simulink model "EV_Truck_Model"  (R2022b)
settings: Solver=FixedStepAuto  StartTime=0  StopTime=26553  FixedStep=0.1  RelTol=1e-3
model workspace (MAT data in the model file):
  ADAS_MaxAccel = 2
  ADAS_MaxDecel = 2.5
  Adas_on_off = 0
  Batt_cap_ah : Simulink.Parameter (value not decoded)
  Batt_rist_r0 : Simulink.Parameter (value not decoded)
  Batt_soc_s0 : Simulink.Parameter (value not decoded)
  Batt_volt_v0 : Simulink.Parameter (value not decoded)
  Motor_eff_100 : Simulink.Parameter (value not decoded)
  Motor_eff_190 : Simulink.Parameter (value not decoded)
  Motor_eff_95 : Simulink.Parameter (value not decoded)
  Motor_rpm_100 : Simulink.Parameter (value not decoded)
  Motor_rpm_190 : Simulink.Parameter (value not decoded)
  Motor_rpm_95 : Simulink.Parameter (value not decoded)
  Motor_torque_pos_100 : Simulink.Parameter (value not decoded)
  Motor_torque_pos_190 : Simulink.Parameter (value not decoded)
  Motor_torque_pos_95 : Simulink.Parameter (value not decoded)
  Motor_trq_190 : Simulink.Parameter (value not decoded)
  Motor_trq_95 : Simulink.Parameter (value not decoded)
  Sim_step = 0.1
  Test_DriveCycle = 0
  Trans_ratio = 6.142
  Veh_cog_fx = 1.69543
  Veh_cog_h = 0.605887
  Veh_cog_rx = 2.11956
  Veh_diff = 6.7
  Veh_whl_crr = 0.01
  Veh_whl_k = 180000
  Veh_whl_radius = 0.35
symbols that are objects in the model workspace (value not decoded): Motor_eff_100, Motor_eff_190, Motor_eff_95, Motor_rpm_100, Motor_rpm_190, Motor_rpm_95, Motor_torque_pos_100, Motor_torque_pos_190, Motor_torque_pos_95, Motor_trq_190, Motor_trq_95
undefined symbols (not defined in the file): Batt_soc_init, canChannel, Elec_aux_sw, Elec_rgn_sw, Power_option, speed, time, Veh_mass
libraries: batteryecm_lib x170, simulink x14, canmsglib x9, canlib x7, autolibshared x5, nesl_utility x4, fl_lib x3, drivingvehiclecontroller x3, hdlsllib x3, sim3dlib x1, sim3dautolib x1, vrlib x1
(part 2 of 11)

== system EV_Truck_Model/Accumulator System ==
  note: Voltage-Capacity Relationship
      | 100% 3.65V
      | 99% 3.4V
      | 98% 3.32V
      | 97% 3.3V
      | Linear
      | 50% 3.2V
      | 20% 3.1V
      | 15% 3.0V
      | 10% 2.8V
      | 5% 2.5V
      | 0% 2.0V
      | Singel Cell Internal Resistance: 3mOhm
      | Parallel Cell Internal Resistance: 0.5mOhm
      | http://hf-gotion.com/products/case5/7.html
  Current : Inport
  2-D Lookup Table : Lookup_n-D  Commented=on  BreakpointsForDimension1=[1:3]  BreakpointsForDimension2=[1:3]  InternalRulePriority=Speed  RndMeth=Simplest
      settings: InputPortMap=u0,u1
  Battery (Table-Based) : batteryecm_lib/Battery (Table-Based)  Tag={'toolbox/physmod/battery/shared_library/m/batteryecm_lib_parts';'Battery__Table_Based_/A123/ALM12V7.xml'}  Commented=through  SOC_vec=[0 0.01 0.02 0.03 0.04 0.05 0.06 0.07 0.08 0.09 0.1 0.11 0.12 0.13 0.14 0.15 0.16 0.17 0.18 0.19 0.2 0.21 0.22 0.23 0.24 0.25 0.26 0.27 0.28 0.29 0.3 0.31 0.32 0.33 0.34 0.35 0.36 0.37 0.38 0.39 0.4 0.41 0.42 0.43 0.44 0.45 0.46 0.47 0.48 0.49 0.5 0.51 0.52 0.53 0.54 0.55 0.56 0.57 0.58 0.59 0.6 0.61 0.62 0.63 0.64 0.65 0.66 0.67 0.68 0.69 0.7 0.71 0.72 0.73 0.74 0.75 0.76 0.77 0.78 0.79 0.8 0.81 0.82 0.83 0.84 0.85 0.86 0.87 0.88 0.89 0.9 0.91 0.92 0.93 0.94 0.95 0.96 0.97 0.98 0.99 1]  T_dependence=simscape.enum.tablebattery.temperature_dependence.yes  prm_dir=simscape.enum.tablebattery.prm_dir.noCurrentDirectionality  T_vec=[0 25 45] degC  V0_mat=[8.05812 7.90952 10.84524;8.40413 8.34439 12.167;8.75015 8.77925 12.48061;9.09617 9.21411 12.63926;9.44219 9.64898 12.66062;9.7882 10.08384 12.66196;10.13422 10.74357 12.71107;10.48024 11.30381 12.78816;10.82626 11.63268 12.79883;11.17301 11.93821 12.78814;11.4915 12.15298 12.76631;11.73964 12.3273 12.75774;11.93281 12.43261 12.76614;12.03376 12.50816 12.77788;12.15804 12.57594 12.79587;12.26092 12.61755 12.81552;12.35763 12.64457 12.83633;12.46264 12.68224 12.84719;12.54135 12.71382 12.85759;12.61973 12.74201 12.87378;12.68064 12.76384 12.89165;12.7273 12.7798 12.90334;12.75019 12.8011 12.91442;12.7795 12.81807 12.92545;12.79476 12.83474 12.93649;12.80199 12.84972 12.94845;12.79988 12.86401 12.96057;12.8064 12.87896 12.97362;12.81314 12.89327 12.9873;12.81905 12.90705 13.00097;12.8231 12.92025 13.01743;12.83144 12.93293 13.03449;12.84056 12.94496 13.05153;12.84748 12.95422 13.06837;12.8514 12.96347 13.08315;12.85351 12.97316 13.09593;12.86138 12.98357 13.10749;12.87252 12.99397 13.11297;12.87348 13.00292 13.1193;12.87448 13.00978 13.12225;12.88062 13.01665 13.12493;12.88615 13.02351 13.1275;12.89358 13.02933 13.12903;12.90102 13.03559 13.13047;12.90646 13.04185 13.1317;12.91023 13.04811 13.13261;12.91373 13.05484 13.1336;12.91916 13.06156 13.13482;12.92679 13.06811 13.13582;12.93442 13.07393 13.13682;12.93761 13.07931 13.13785;12.93879 13.08459 13.14019;12.94047 13.08888 13.1426;12.94372 13.09316 13.14505;12.94697 13.09745 13.14506;12.95275 13.10191 13.14506;12.95871 13.10663 13.14507;12.96447 13.11149 13.14537;12.97023 13.11625 13.14712;12.97671 13.12077 13.14887;12.98396 13.1253 13.15078;12.9912 13.12947 13.15349;12.99846 13.13339 13.15917;13.00592 13.13718 13.16486;13.0098 13.142 13.17126;13.01315 13.14683 13.1789;13.01642 13.15338 13.18676;13.0194 13.1606 13.19727;13.0225 13.16782 13.20775;13.03012 13.17504 13.21901;13.03927 13.18103 13.23221;13.04842 13.18612 13.24601;13.05758 13.19115 13.25559;13.06673 13.19583 13.26268;13.07323 13.20057 13.26837;13.07926 13.20546 13.27148;13.08529 13.21036 13.27459;13.09132 13.21551 13.27817;13.10058 13.22106 13.28185;13.11119 13.22814 13.28528;13.12181 13.23521 13.28448;13.13279 13.24229 13.2834;13.14332 13.24921 13.28542;13.14826 13.25386 13.28855;13.15276 13.25892 13.29055;13.15658 13.26397 13.29097;13.15965 13.26903 13.29534;13.1637 13.27459 13.29849;13.16904 13.2803 13.29921;13.17556 13.28425 13.29987;13.18215 13.2873 13.30304;13.18702 13.29077 13.30748;13.18906 13.29423 13.31134;13.19472 13.29701 13.31689;13.20216 13.30359 13.32162;13.20682 13.31175 13.33363;13.21832 13.31809 13.34341;13.22486 13.34117 13.3682;13.25687 13.37591 13.4231;13.3584 13.50696 13.59952;13.73658 14.69171 14.24081] V  V0_vec=[7.90952 8.34439 8.77925 9.21411 9.64898 10.08384 10.74357 11.30381 11.63268 11.93821 12.15298 12.3273 12.43261 12.50816 12.57594 12.61755 12.64457 12.68224 12.71382 12.74201 12.76384 12.7798 12.8011 12.81807 12.83474 12.84972 12.86401 12.87896 12.89327 12.90705 12.92025 12.93293 12.94496 12.95422 12.96347 12.97316 12.98357 12.99397 13.00292 13.00978 13.01665 13.02351 13.02933 13.03559 13.04185 13.04811 13.05484 13.06156 13.06811 13.07393 13.07931 13.08459 13.08888 13.09316 13.09745 13.10191 13.10663 13.11149 13.11625 13.12077 13.1253 13.12947 13.13339 13.13718 13.142 13.14683 13.15338 13.1606 13.16782 13.17504 13.18103 13.18612 13.19115 13.19583 13.20057 13.20546 13.21036 13.21551 13.22106 13.22814 13.23521 13.24229 13.24921 13.25386 13.25892 13.26397 13.26903 13.27459 13.2803 13.28425 13.2873 13.29077 13.29423 13.29701 13.30359 13.31175 13.31809 13.34117 13.37591 13.50696 14.69171] V  V_range=[9 Inf] V  R0_mat=[0.24852 0.16316 0.37407;0.27167 0.15014 0.44119;0.29483 0.13711 0.39874;0.31798 0.12409 0.33945;0.34114 0.11107 0.253;0.36429 0.09804 0.17297;0.38744 0.09898 0.137;0.4106 0.09406 0.11837;0.43375 0.07751 0.0969;0.45706 0.07197 0.08022;0.47423 0.06587 0.06407;0.47611 0.06364 0.05484;0.46604 0.05937 0.05112;0.43592 0.0557 0.04879;0.41518 0.05497 0.04766;0.39502 0.05305 0.04722;0.3785 0.05058 0.04739;0.36725 0.05063 0.04645;0.34844 0.05036 0.04531;0.33707 0.04999 0.0448;0.32097 0.04932 0.045;0.30505 0.04837 0.04454;0.28497 0.04827 0.04408;0.2684 0.04798 0.04361;0.25118 0.04766 0.04314;0.23446 0.04729 0.04289;0.21678 0.04694 0.04266;0.20301 0.0471 0.04269;0.19098 0.04724 0.0429;0.1805 0.04736 0.0431;0.17153 0.04745 0.04377;0.16488 0.04751 0.04456;0.15901 0.04755 0.04534;0.15295 0.04741 0.04605;0.14764 0.04727 0.04643;0.1423 0.04726 0.04659;0.13996 0.04731 0.04663;0.13837 0.04736 0.04628;0.13485 0.04731 0.0463;0.13134 0.04714 0.04596;0.12898 0.04697 0.04558;0.1265 0.0468 0.04516;0.12564 0.04664 0.04461;0.12479 0.04662 0.04405;0.1235 0.04659 0.04344;0.12161 0.04657 0.04278;0.11961 0.04658 0.04214;0.11837 0.04659 0.04165;0.11809 0.04657 0.04112;0.11781 0.04651 0.0406;0.11651 0.04644 0.0401;0.11476 0.04636 0.03973;0.11322 0.04622 0.03938;0.11237 0.04607 0.03905;0.11152 0.04593 0.03846;0.11122 0.04582 0.03787;0.11069 0.04573 0.03729;0.11008 0.04565 0.03668;0.10947 0.04556 0.03617;0.10916 0.04546 0.03567;0.10918 0.04535 0.03524;0.10919 0.04524 0.03503;0.10922 0.04511 0.03515;0.10933 0.04499 0.03527;0.10866 0.04502 0.03552;0.10787 0.04505 0.03591;0.10706 0.04519 0.03633;0.10611 0.04538 0.03685;0.10519 0.04556 0.03735;0.10529 0.04574 0.03794;0.10605 0.04585 0.03887;0.10682 0.04586 0.04006;0.10758 0.04586 0.0408;0.10835 0.04585 0.04126;0.10839 0.04585 0.04147;0.10829 0.04585 0.04134;0.10819 0.04586 0.0412;0.10809 0.0459 0.04113;0.10886 0.046 0.04108;0.10997 0.04618 0.041;0.11107 0.04637 0.04018;0.11233 0.04655 0.03922;0.11356 0.04673 0.03886;0.11359 0.04676 0.03865;0.11341 0.04683 0.03842;0.11294 0.04689 0.03823;0.11231 0.04695 0.03846;0.1122 0.04704 0.03796;0.11241 0.04714 0.03717;0.11291 0.04696 0.03641;0.11346 0.0466 0.03639;0.11363 0.04626 0.0365;0.11258 0.04592 0.0362;0.11218 0.04538 0.0359;0.11216 0.04507 0.03525;0.11038 0.04454 0.03533;0.11007 0.04279 0.03431;0.1059 0.04194 0.03432;0.09933 0.03873 0.03411;0.09302 0.03651 0.038;0.07895 0.07068 0.04545] Ohm  R0_vec=[0.16316 0.15014 0.13711 0.12409 0.11107 0.09804 0.09898 0.09406 0.07751 0.07197 0.06587 0.06364 0.05937 0.0557 0.05497 0.05305 0.05058 0.05063 0.05036 0.04999 0.04932 0.04837 0.04827 0.04798 0.04766 0.04729 0.04694 0.0471 0.04724 0.04736 0.04745 0.04751 0.04755 0.04741 0.04727 0.04726 0.04731 0.04736 0.04731 0.04714 0.04697 0.0468 0.04664 0.04662 0.04659 0.04657 0.04658 0.04659 0.04657 0.04651 0.04644 0.04636 0.04622 0.04607 0.04593 0.04582 0.04573 0.04565 0.04556 0.04546 0.04535 0.04524 0.04511 0.04499 0.04502 0.04505 0.04519 0.04538 0.04556 0.04574 0.04585 0.04586 0.04586 0.04585 0.04585 0.04585 0.04586 0.0459 0.046 0.04618 0.04637 0.04655 0.04673 0.04676 0.04683 0.04689 0.04695 0.04704 0.04714 0.04696 0.0466 0.04626 0.04592 0.04538 0.04507 0.04454 0.04279 0.04194 0.03873 0.03651 0.07068] Ohm  R0_dis_mat=[.0117, .0085, .009; .011, .0085, .009; .0114, .0087, .0092; .0107, .0082, .0088; .0107, .0083, .0091; .0113, .0085, .0089; .0116, .0085, .0089] % Parameter not set Ohm  R0_dis_vec=[.0085, .0085, .0087, .0082, .0083, .0085, .0085] % Parameter not set Ohm  R0_ch_mat=[.0117, .0085, .009; .011, .0085, .009; .0114, .0087, .0092; .0107, .0082, .0088; .0107, .0083, .0091; .0113, .0085, .0089; .0116, .0085, .0089] % Parameter not set Ohm  R0_ch_vec=[.0085, .0085, .0087, .0082, .0083, .0085, .0085] % Parameter not set Ohm  AH=4.911 hr*A  prm_leak=simscape.enum.tablebattery.prm_leak.disabled  Rleak_vec=[8000, 7000, 6000] % Parameter not set Ohm  Rleak=7e3 % Parameter not set Ohm  extrapolation_option=simscape.enum.extrapolation.nearest  SOC_port=simscape.enum.tablebattery.enable.no  prm_dyn=simscape.enum.tablebattery.prm_dyn.off  R1_mat=[.0109, .0029, .0013; .0069, .0024, .0012; .0047, .0026, .0013; .0034, .0016, .001; .0033, .0023, .0014; .0033, .0018, .0011; .0028, .0017, .0011] % Parameter not set Ohm  R1_vec=[.0029, .0024, .0026, .0016, .0023, .0018, .0017] % Parameter not set Ohm  tau1_mat=[20, 36, 39; 31, 45, 39; 109, 105, 61; 36, 29, 26; 59, 77, 67; 40, 33, 29; 25, 39, 33] % Parameter not set s  tau1_vec=[36, 45, 105, 29, 77, 33, 39] % Parameter not set s  R2_mat=[.0109, .0029, .0013; .0069, .0024, .0012; .0047, .0026, .0013; .0034, .0016, .001; .0033, .0023, .0014; .0033, .0018, .0011; .0028, .0017, .0011] % Parameter not set Ohm  R2_vec=[.0029, .0024, .0026, .0016, .0023, .0018, .0017] % Parameter not set Ohm  tau2_mat=[20, 36, 39; 31, 45, 39; 109, 105, 61; 36, 29, 26; 59, 77, 67; 40, 33, 29; 25, 39, 33] % Parameter not set s  tau2_vec=[36, 45, 105, 29, 77, 33, 39] % Parameter not set s  R3_mat=[.0109, .0029, .0013; .0069, .0024, .0012; .0047, .0026, .0013; .0034, .0016, .001; .0033, .0023, .0014; .0033, .0018, .0011; .0028, .0017, .0011] % Parameter not set Ohm  R3_vec=[.0029, .0024, .0026, .0016, .0023, .0018, .0017] % Parameter not set Ohm  tau3_mat=[20, 36, 39; 31, 45, 39; 109, 105, 61; 36, 29, 26; 59, 77, 67; 40, 33, 29; 25, 39, 33] % Parameter not set s  tau3_vec=[36, 45, 105, 29, 77, 33, 39] % Parameter not set s  R4_mat=[.0109, .0029, .0013; .0069, .0024, .0012; .0047, .0026, .0013; .0034, .0016, .001; .0033, .0023, .0014; .0033, .0018, .0011; .0028, .0017, .0011] % Parameter not set Ohm  R4_vec=[.0029, .0024, .0026, .0016, .0023, .0018, .0017] % Parameter not set Ohm  tau4_mat=[20, 36, 39; 31, 45, 39; 109, 105, 61; 36, 29, 26; 59, 77, 67; 40, 33, 29; 25, 39, 33] % Parameter not set s  tau4_vec=[36, 45, 105, 29, 77, 33, 39] % Parameter not set s  R5_mat=[.0109, .0029, .0013; .0069, .0024, .0012; .0047, .0026, .0013; .0034, .0016, .001; .0033, .0023, .0014; .0033, .0018, .0011; .0028, .0017, .0011] % Parameter not set Ohm  R5_vec=[.0029, .0024, .0026, .0016, .0023, .0018, .0017] % Parameter not set Ohm  tau5_mat=[20, 36, 39; 31, 45, 39; 109, 105, 61; 36, 29, 26; 59, 77, 67; 40, 33, 29; 25, 39, 33] % Parameter not set s  tau5_vec=[36, 45, 105, 29, 77, 33, 39] % Parameter not set s  prm_fade=simscape.enum.tablebattery.prm_fade.tableN  N0=100 % Parameter not set  dV0=0 % Parameter not set  dR0=0 % Parameter not set  dAH=0 % Parameter not set  dRleak=0 % Parameter not set  dR1=0 % Parameter not set  dR2=0 % Parameter not set  dR3=0 % Parameter not set  dR4=0 % Parameter not set  dR5=0 % Parameter not set  N0vec=[1 76 151 226 301 376 451 526 601 676 751 826 901 976 1051 1126 1201 1276 1351 1426 1501 1576 1651 1726 1801 1876 1951 2026 2101 2176 2251 2326 2401 2476 2551 2626 2701 2776 2851 2926 3001 3076 3151 3226 3301 3376 3451 3526 3601 3676 3751 3826 3901 3976 4051 4126 4201 4276 4351 4426 4501 4576 4651 4726 4801 4876 4951 5026 5101 5176 5251 5326 5401 5476 5551 5626 5701 5776 5851 5926 6001 6076 6151 6226 6301 6376 6451 6526 6601 6676 6751 6826 6901 6976 7051 7126 7201 7276 7351]  Tfadevec=[298.15, 323.15] % Parameter not set K  dV0vec=[0 -2.2983 -4.5967 -6.895 -8.189 -8.4451 -8.8012 -9.0094 -9.1038 -9.1836 -9.2343 -9.282 -9.3297 -9.3564 -9.3673 -9.3782 -9.3891 -9.402 -9.4162 -9.4327 -9.4491 -9.4624 -9.4766 -9.4917 -9.4989 -9.5047 -9.5093 -9.5145 -9.5202 -9.5259 -9.531 -9.5361 -9.5412 -9.5463 -9.5514 -9.557 -9.5622 -9.5672 -9.5722 -9.5771 -9.5822 -9.5878 -9.5934 -9.599 -9.6046 -9.6114 -9.6185 -9.6256 -9.6327 -9.6397 -9.6463 -9.651 -9.6557 -9.6605 -9.6652 -9.67 -9.6747 -9.6803 -9.6857 -9.6908 -9.6959 -9.701 -9.7064 -9.7127 -9.7189 -9.7252 -9.7314 -9.738 -9.7446 -9.7511 -9.7577 -9.7643 -9.767 -9.7695 -9.772 -9.7748 -9.7798 -9.7848 -9.7896 -9.7948 -9.8002 -9.8056 -9.811 -9.8162 -9.8181 -9.8205 -9.8232 -9.8259 -9.8291 -9.836 -9.843 -9.8499 -9.8569 -9.8644 -9.872 -9.8797 -9.8867 -9.8926 -9.8986]  dR0vec=[0 0 0 0 0 0 0 0 0 0 0 0 0 0 0 0 0 0 0 0 0 0 0 0 0 0 0 0 0 0 0 0 0 0 0 0 0 0 0 0 0 0 0 0 0 0 0 0 0 0 0 0 0 0 0 0 0 0 0 0 0 0 0 0 0 0 0 0 0 0 0 0 0 0 0 0 0 0 0 0 0 0 0 0 0 0 0 0 0 0 0 0 0 0 0 0 0 0 0] % Parameter assumed  dAHvec=[0 -0.285 -0.57 -0.855 -1.14 -1.427 -1.826 -2.226 -2.625 -2.962 -3.266 -3.569 -3.873 -4.157 -4.409 -4.662 -4.914 -5.167 -5.421 -5.719 -6.017 -6.316 -6.632 -6.968 -7.304 -7.613 -7.858 -8.103 -8.349 -8.589 -8.804 -9.02 -9.236 -9.452 -9.668 -9.906 -10.145 -10.384 -10.623 -10.862 -11.083 -11.291 -11.499 -11.707 -11.914 -12.118 -12.3 -12.482 -12.664 -12.846 -13.015 -13.14 -13.265 -13.39 -13.515 -13.64 -13.766 -13.913 -14.061 -14.21 -14.358 -14.506 -14.664 -14.846 -15.027 -15.209 -15.391 -15.582 -15.772 -15.963 -16.154 -16.345 -16.424 -16.497 -16.569 -16.65 -16.796 -16.943 -17.09 -17.252 -17.423 -17.594 -17.765 -17.93 -17.987 -18.044 -18.1 -18.157 -18.226 -18.373 -18.52 -18.668 -18.815 -18.974 -19.134 -19.294 -19.438 -19.562 -19.686]  dRleakvec=[0, 0, 0] % Parameter not set  dR1vec=[0, 0, 0] % Parameter not set  dR2vec=[0, 0, 0] % Parameter not set  dR3vec=[0, 0, 0] % Parameter not set  dR4vec=[0, 0, 0] % Parameter not set  dR5vec=[0, 0, 0] % Parameter not set  dV0mat=[0, 0; 0, 0; 0, 0] % Parameter not set  dR0mat=[0, 0; 0, 0; 0, 0] % Parameter not set  dAHmat=[0, 0; 0, 0; 0, 0] % Parameter not set  dRleakmat=[0, 0; 0, 0; 0, 0] % Parameter not set  dR1mat=[0, 0; 0, 0; 0, 0] % Parameter not set  dR2mat=[0, 0; 0, 0; 0, 0] % Parameter not set  dR3mat=[0, 0; 0, 0; 0, 0] % Parameter not set  dR4mat=[0, 0; 0, 0; 0, 0] % Parameter not set  dR5mat=[0, 0; 0, 0; 0, 0] % Parameter not set  prm_age_modeling=simscape.enum.tablebattery.prm_age_modeling.equation  storage_dt_age_vec=[0] % Parameter not set d  storage_T_age_vec=[273] % Parameter not set K  prm_age_OCV=simscape.enum.tablebattery.prm_age_OCV.OCV  OCV_age=0.9 % Parameter not set  SOC_age=0.6 % Parameter not set  prm_age_resistance=simscape.enum.tablebattery.prm_age.disabled  OCV_scaling_age_resistance=2.2134e6 % Parameter not set  OCV_offset_age_resistance=1.632e6 % Parameter not set  temp_exp_age_resistance=0.515833569 % Parameter not set V  t_exp_age_resistance=0.75 % Parameter not set  T_age_vec_resistance=[273.15, 298.15, 323.15] % Parameter not set K  dt_age_vec_resistance=[90, 180, 270, 360] % Parameter not set d  dR0_age_vec=[0, 0, 0] % Parameter not set  t_meas_dR0_age=100 % Parameter not set d  dR0_age_mat=[0, 0, 0; 0, 0, 0; 0, 0, 0; 0, 0, 0] % Parameter not set  prm_age_capacity=simscape.enum.tablebattery.prm_age.disabled  OCV_scaling_age_capacity=1.5097e07 % Parameter not set  OCV_offset_age_capacity=8.3625e06 % Parameter not set  temp_exp_age_capacity=0.6011 % Parameter not set V  t_exp_age_capacity=0.75 % Parameter not set  T_age_vec_capacity=[273.15, 298.15, 323.15] % Parameter not set K  dt_age_vec_capacity=[90, 180, 270, 360] % Parameter not set d  dAH_age_vec=[0, 0, 0] % Parameter not set  t_meas_dAH_age=100 % Parameter not set d  dAH_age_mat=[0, 0, 0; 0, 0, 0; 0, 0, 0; 0, 0, 0] % Parameter not set  thermal_port=simscape.enum.thermaleffects.omit  temperature=298.15 % Parameter not set K  thermal_mass=756 % Parameter assumed J/K  i_specify=off  i_priority=None  i=0 A  i_nominal_specify=off  i_nominal_unit=A  i_nominal_value=1  v_specify=off  v_priority=None  v=0 V  v_nominal_specify=off  v_nominal_unit=V  v_nominal_value=1  stateOfCharge_specify=off  stateOfCharge_priority=High  stateOfCharge=1  stateOfCharge_nominal_specify=off  stateOfCharge_nominal_unit=1  stateOfCharge_nominal_value=1  num_cycles_specify=off  num_cycles_priority=High  num_cycles=0  num_cycles_nominal_specify=off  num_cycles_nominal_unit=1  num_cycles_nominal_value=1  cell_temperature_specify=off  cell_temperature_priority=High  cell_temperature=298.15 K  cell_temperature_nominal_specify=off  cell_temperature_nominal_unit=K  cell_temperature_nominal_value=1
      settings: AttributesFormatString=A123:ALM12V7  InternalSimscapePortConfiguration="{\"Bottom\":[],\"Left\":[{\"id\":\"p\",\"label\":\"+\",\"type\":\"foundation.electrical.electrical\"}],\"Right\":[{\"id\":\"n\",\"label\":\"-\",\"type\":\"foundation.electrical.electrical\"}],\"Top\":[]}"
  Battery Pack : Subsystem
  Battery1 : batteryecm_lib/Battery (Table-Based)  Commented=on  SOC_vec=Batt_soc_s0  T_dependence=simscape.enum.tablebattery.temperature_dependence.no  prm_dir=simscape.enum.tablebattery.prm_dir.noCurrentDirectionality  T_vec=[293] K  V0_mat=[2, 3, 3.2, 3.25, 3.25, 3.3, 3.3, 3.3, 3.35, 3.5] V  V0_vec=Batt_volt_v0 V  V_range=[0, inf] V  R0_mat=[15] mOhm  R0_vec=Batt_rist_r0 mOhm  R0_dis_mat=[.0117, .0085, .009; .011, .0085, .009; .0114, .0087, .0092; .0107, .0082, .0088; .0107, .0083, .0091; .0113, .0085, .0089; .0116, .0085, .0089] Ohm  R0_dis_vec=[.0085, .0085, .0087, .0082, .0083, .0085, .0085] Ohm  R0_ch_mat=[.0117, .0085, .009; .011, .0085, .009; .0114, .0087, .0092; .0107, .0082, .0088; .0107, .0083, .0091; .0113, .0085, .0089; .0116, .0085, .0089] Ohm  R0_ch_vec=[.0085, .0085, .0087, .0082, .0083, .0085, .0085] Ohm  AH=Batt_cap_ah A*hr  prm_leak=simscape.enum.tablebattery.prm_leak.disabled  Rleak_vec=[8000, 7000, 6000] Ohm  Rleak=7e3 Ohm  extrapolation_option=simscape.enum.extrapolation.nearest  SOC_port=simscape.enum.tablebattery.enable.no  prm_dyn=simscape.enum.tablebattery.prm_dyn.off  R1_mat=[.0109, .0029, .0013; .0069, .0024, .0012; .0047, .0026, .0013; .0034, .0016, .001; .0033, .0023, .0014; .0033, .0018, .0011; .0028, .0017, .0011] Ohm  R1_vec=[.0029, .0024, .0026, .0016, .0023, .0018, .0017] Ohm  tau1_mat=[20, 36, 39; 31, 45, 39; 109, 105, 61; 36, 29, 26; 59, 77, 67; 40, 33, 29; 25, 39, 33] s  tau1_vec=[36, 45, 105, 29, 77, 33, 39] s  R2_mat=[.0109, .0029, .0013; .0069, .0024, .0012; .0047, .0026, .0013; .0034, .0016, .001; .0033, .0023, .0014; .0033, .0018, .0011; .0028, .0017, .0011] Ohm  R2_vec=[.0029, .0024, .0026, .0016, .0023, .0018, .0017] Ohm  tau2_mat=[20, 36, 39; 31, 45, 39; 109, 105, 61; 36, 29, 26; 59, 77, 67; 40, 33, 29; 25, 39, 33] s  tau2_vec=[36, 45, 105, 29, 77, 33, 39] s  R3_mat=[.0109, .0029, .0013; .0069, .0024, .0012; .0047, .0026, .0013; .0034, .0016, .001; .0033, .0023, .0014; .0033, .0018, .0011; .0028, .0017, .0011] Ohm  R3_vec=[.0029, .0024, .0026, .0016, .0023, .0018, .0017] Ohm  tau3_mat=[20, 36, 39; 31, 45, 39; 109, 105, 61; 36, 29, 26; 59, 77, 67; 40, 33, 29; 25, 39, 33] s  tau3_vec=[36, 45, 105, 29, 77, 33, 39] s  R4_mat=[.0109, .0029, .0013; .0069, .0024, .0012; .0047, .0026, .0013; .0034, .0016, .001; .0033, .0023, .0014; .0033, .0018, .0011; .0028, .0017, .0011] Ohm  R4_vec=[.0029, .0024, .0026, .0016, .0023, .0018, .0017] Ohm  tau4_mat=[20, 36, 39; 31, 45, 39; 109, 105, 61; 36, 29, 26; 59, 77, 67; 40, 33, 29; 25, 39, 33] s  tau4_vec=[36, 45, 105, 29, 77, 33, 39] s  R5_mat=[.0109, .0029, .0013; .0069, .0024, .0012; .0047, .0026, .0013; .0034, .0016, .001; .0033, .0023, .0014; .0033, .0018, .0011; .0028, .0017, .0011] Ohm  R5_vec=[.0029, .0024, .0026, .0016, .0023, .0018, .0017] Ohm  tau5_mat=[20, 36, 39; 31, 45, 39; 109, 105, 61; 36, 29, 26; 59, 77, 67; 40, 33, 29; 25, 39, 33] s  tau5_vec=[36, 45, 105, 29, 77, 33, 39] s  prm_fade=simscape.enum.tablebattery.prm_fade.disabled  N0=100  dV0=0  dR0=0  dAH=0  dRleak=0  dR1=0  dR2=0  dR3=0  dR4=0  dR5=0  N0vec=[100, 200, 300]  Tfadevec=[298.15, 323.15] K  dV0vec=[0, 0, 0]  dR0vec=[0, 0, 0]  dAHvec=[0, 0, 0]  dRleakvec=[0, 0, 0]  dR1vec=[0, 0, 0]  dR2vec=[0, 0, 0]  dR3vec=[0, 0, 0]  dR4vec=[0, 0, 0]  dR5vec=[0, 0, 0]  dV0mat=[0, 0; 0, 0; 0, 0]  dR0mat=[0, 0; 0, 0; 0, 0]  dAHmat=[0, 0; 0, 0; 0, 0]  dRleakmat=[0, 0; 0, 0; 0, 0]  dR1mat=[0, 0; 0, 0; 0, 0]  dR2mat=[0, 0; 0, 0; 0, 0]  dR3mat=[0, 0; 0, 0; 0, 0]  dR4mat=[0, 0; 0, 0; 0, 0]  dR5mat=[0, 0; 0, 0; 0, 0]  prm_age_modeling=simscape.enum.tablebattery.prm_age_modeling.equation  storage_dt_age_vec=[0] d  storage_T_age_vec=[273] K  prm_age_OCV=simscape.enum.tablebattery.prm_age_OCV.OCV  OCV_age=0.9  SOC_age=0.6  prm_age_resistance=simscape.enum.tablebattery.prm_age.disabled  OCV_scaling_age_resistance=2.2134e6  OCV_offset_age_resistance=1.632e6  temp_exp_age_resistance=0.515833569 V  t_exp_age_resistance=0.75  T_age_vec_resistance=[273.15, 298.15, 323.15] K  dt_age_vec_resistance=[90, 180, 270, 360] d  dR0_age_vec=[0, 0, 0]  t_meas_dR0_age=100 d  dR0_age_mat=[0, 0, 0; 0, 0, 0; 0, 0, 0; 0, 0, 0]  prm_age_capacity=simscape.enum.tablebattery.prm_age.disabled  OCV_scaling_age_capacity=1.5097e07  OCV_offset_age_capacity=8.3625e06  temp_exp_age_capacity=0.6011 V  t_exp_age_capacity=0.75  T_age_vec_capacity=[273.15, 298.15, 323.15] K  dt_age_vec_capacity=[90, 180, 270, 360] d  dAH_age_vec=[0, 0, 0]  t_meas_dAH_age=100 d  dAH_age_mat=[0, 0, 0; 0, 0, 0; 0, 0, 0; 0, 0, 0]  thermal_port=simscape.enum.thermaleffects.omit  temperature=298.15 K  thermal_mass=100 J/K  i_specify=off  i_priority=None  i=0 A  i_nominal_specify=off  i_nominal_unit=A  i_nominal_value=1  v_specify=off  v_priority=None  v=0 V  v_nominal_specify=off  v_nominal_unit=V  v_nominal_value=1  stateOfCharge_specify=on  stateOfCharge_priority=High  stateOfCharge=Batt_soc_init  stateOfCharge_nominal_specify=off  stateOfCharge_nominal_unit=1  stateOfCharge_nominal_value=1  num_cycles_specify=off  num_cycles_priority=High  num_cycles=0  num_cycles_nominal_specify=off  num_cycles_nominal_unit=1  num_cycles_nominal_value=1  cell_temperature_specify=off  cell_temperature_priority=High  cell_temperature=298.15 K  cell_temperature_nominal_specify=off  cell_temperature_nominal_unit=K  cell_temperature_nominal_value=1
      settings: InternalSimscapePortConfiguration="{\"Bottom\":[],\"Left\":[{\"id\":\"p\",\"label\":\"+\",\"type\":\"foundation.electrical.electrical\"}],\"Right\":[{\"id\":\"n\",\"label\":\"-\",\"type\":\"foundation.electrical.electrical\"}],\"Top\":[]}"
  Fusible Link : Subsystem
  Power Calculator : Subsystem
      settings: PortSchema="{\"entries\":[{\"content\":{\"sides\":[{\"content\":{\"connectorIds\":[\"In1\"]},\"type\":\"ConnectorPlacement.EquallySpacedRectSide\",\"uuid\":\"d8d02989-bfd1-459d-a417-26b1aef8d33a\"},{\"content\":{\"connectorIds\":[\"Out1\",\"Out2\",\"Out3\"],\"side\":\"RIGHT\"},\"type\":\"ConnectorPlacement.EquallySpacedRectSide\",\"uuid\":\"a790ec78-e78f-4679-acdd-9e45889e5bd0\"},{\"content\":{\"connectorIds\":[\"In2\"],\"side\":\"TOP\"},\"type\":\"ConnectorPlacement.EquallySpacedRectSide\",\"uuid\":\"d5690f93-674f-4683-8af2-fe1cf051e81a\"}]},\"type\":\"ConnectorPlacement.EquallySpacedConnector\",\"uuid\":\"0a429913-83d6-4bb6-80aa-ea0e3c9bfed8\"}],\"packageUris\":[\"http://schema.mathworks.com/mf0/Connector/R2020b\"],\"version\":\"1.0\"}"
  Scope : Scope  NumInputPorts=5
  Voltage : Outport
  SOC : Outport  Port=2
  wires:
  Current/1 -> Fusible Link/1(In1)  "Battery_Current(A)"
  [SOC] -> SOC/1, Scope/2  "Battery_SOC(%)"
  Power Calculator/1(Ampacity Consumption) -> Scope/3  "Battery_P_consumed(Ah)"
  Battery Pack/1(VOLT) -> Power Calculator/2(VOLT), Scope/1, Voltage/1
  Power Calculator/2(Power) -> Scope/4  "Battery_P_output(kW)"
  Fusible Link/1(Out1) -> Battery Pack/1(CURR), Power Calculator/1(Current)
  Power Calculator/3(Power Consumption) -> Scope/5  "Battery_P_consumed(kWh)"

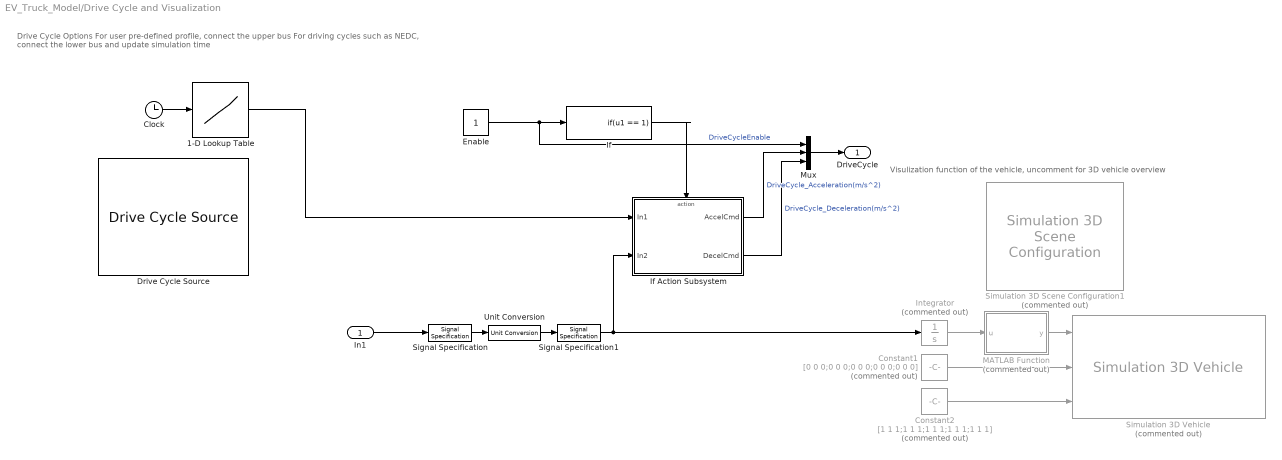
== system EV_Truck_Model/Drive Cycle and Visualization ==
  note: Visulization function of the vehicle, uncomment for 3D vehicle overview
  note: Drive Cycle Options
      | For user pre-defined profile, connect the upper bus
      | For driving cycles such as NEDC, connect the lower bus and update simulation time
  In1 : Inport
  1-D Lookup Table : Lookup_n-D  NumberOfTableDimensions=1  BreakpointsForDimension1=time  Table=speed  InternalRulePriority=Speed  RndMeth=Simplest
  Clock : Clock
  Constant1 : Constant  Commented=on  Value=[0 0 0;0 0 0;0 0 0;0 0 0;0 0 0]
  Constant2 : Constant  Commented=on  Value=[1 1 1;1 1 1;1 1 1;1 1 1;1 1 1]
  Drive Cycle Source : autolibshared/Drive Cycle Source  cycleVar=FTP75  fileVar=cycleFTP75.mat  tfinal="2474  seconds"  cycleRepeat=off  outAccPort=off  outGearPort=off  gearList=No gear data  t_wot1=5  xdot_woto=0  xdot_wot1=30  t_wot2=20  xdot_wot2=0  t_wotend=30  srcUnit=m/s  outUnit=m/s  srcAccUnit=m/s/s  outAccUnit=m/s^2  dt=0  aMode=1  faultOption=off  velBnd=2  velBndUnit=mph  inUnit=m/s  timeBnd=1  failOption=off  stopSim=off  maxFaultCnt=10  maxFaultTime=2  maxTotFaultTime=15  traceOption=off  dtTrace=1  traceWindow=10  lastDCname=FTP75  lastOutUnit=mph  lastDT=0  lastTB=1  lastSB=2  forceCalcBound=off
  Enable : Constant
  If : If  IfExpression=u1 == 1  ShowElse=off
  If Action Subsystem : Subsystem  TreatAsAtomicUnit=on
  Integrator : Integrator  Commented=on
  MATLAB Function : MATLAB Function  Commented=on  TreatAsAtomicUnit=on
  Mux : Mux  Inputs=3
  Signal Specification : SignalSpecification  Unit=km/hr
  Signal Specification1 : SignalSpecification  Unit=m/s
  Simulation 3D Scene Configuration1 : sim3dlib/Simulation 3D Scene Configuration  Priority=0  Commented=on  ProjectFormat=Default Scenes  SceneDesc=Straight road  ProjectName=C:\Program Files\MATLAB\R2022b\toolbox\shared\sim3d_projects\automotive_project\UE4\WindowsNoEditor\VehicleSimulation.exe  ScenePath=/Game/Maps/HwStrght  EnableOpenDRIVE=off  vehTagList={'Scene Origin';'SimulinkVehicle1'}  vehTag=SimulinkVehicle1  OpVisEn=off  Ts=.05  EnableWindow=on  EnableRemoteAccess=off  EnableWeather=off  SunAltitude=40.0  SunAzimuth=90  clouds=10  wind=1  fog=0  rain=0  EnableGeospatial=off  OriginHeight=200  OriginLatitude=40.744652  OriginLongitude=-73.988864  MapStyle=Aerial  AdditionalAssetIDs=[]  UseAdvancedSunSky=off  SolarTime=11  TimeZone=-5  Day=21  Month=9  Year=2022  UseDaylightSavingTime=on  DSTStartDay=10  DSTStartMonth=3  DSTEndDay=3  DSTEndMonth=11  DSTSwitchHour=2  sensorTag=MainCamera1  sensorId=1  sensorName=MainCamera1  mountLoc=Origin  offsetFlag=off  tmountOffset=[0, 0, 0]  rmountOffset=[0, 0, 0]  HorizontalResolution=1280  VerticalResolution=720  HorizontalFOV=60  mountPoint=[0 0 0]  mountOrientation=[0 0 0]  aMode=2  ID=1  GeoTrigger=Inactive
      settings: LibrarySourceBlock=vdynlib/Vehicle Scenarios/Sim3D/Sim3D Core/Simulation 3D Scene Configuration
  Simulation 3D Vehicle : sim3dautolib/Simulation 3D Vehicle  Priority=-1  Commented=on  PassVehMesh=Box truck  MeshPath=/MathWorksSimulation/Vehicles/Muscle/Meshes/SK_MuscleCar.SK_MuscleCar  VehColor=White  ActorName=SimulinkVehicle1  VehLightsControl=off  HeadlightColor=[ 1, 1, 1 ]  HighBeamIntensity=100000  LowBeamIntensity=60000  HighBeamConeAngle=1.22  LowBeamConeAngle=1.22  LeftHeadlightOrientation=[ 0, 0 ]  RightHeadlightOrientation=[ 0, 0 ]  BrakelightIntensity=500  ReverselightIntensity=500  SignallightIntensity=500  SignallightPeriod=1  SignalPulseWidth=50  Translation=zeros( 5, 3 )  Rotation=zeros( 5, 3 )  Scale=ones( 5, 3 )  SampleTime=-1  ActorType=SimulinkVehicle  ID=1  aMode=2  ActorTag=SimulinkVehicle1
      settings: LibrarySourceBlock=vdynlib/Vehicle Scenarios/Sim3D/Sim3D Vehicle/Components/Simulation 3D Vehicle
  Unit Conversion : UnitConversion
  DriveCycle : Outport
  wires:
  Constant1/1 -> Simulation 3D Vehicle/2
  Constant2/1 -> Simulation 3D Vehicle/3
  MATLAB Function/1(y) -> Simulation 3D Vehicle/1
  Signal Specification1/1 -> Integrator/1, If Action Subsystem/2(In2)
  Integrator/1 -> MATLAB Function/1(u)
  Enable/1 -> Mux/1, If/1  "DriveCycleEnable"
  1-D Lookup Table/1 -> If Action Subsystem/1(In1)
  If/1 -> If Action Subsystem/Action
  If Action Subsystem/1(AccelCmd) -> Mux/2  "DriveCycle_Acceleration(m/s^2)"
  If Action Subsystem/2(DecelCmd) -> Mux/3  "DriveCycle_Deceleration(m/s^2)"
  Mux/1 -> DriveCycle/1
  Unit Conversion/1 -> Signal Specification1/1
  Signal Specification/1 -> Unit Conversion/1
  In1/1 -> Signal Specification/1
  Clock/1 -> 1-D Lookup Table/1

== system EV_Truck_Model/MCU and Motor System ==
  TrqCmd : Inport
  Voltage : Inport  Port=2
  Motor_RPM : Inport  Port=3
  Motor Torque Mapping and MCU Limiter : Subsystem
  Power and Efficiency Estimator : Subsystem
  Terminator : Terminator
  Terminator1 : Terminator
  Terminator2 : Terminator
  Torque : Outport
  TrqLimit : Outport  Port=2
  Current : Outport  Port=3
  wires:
  Motor_RPM/1 -> Motor Torque Mapping and MCU Limiter/2(Motor_RPM), Power and Efficiency Estimator/3(Motor_RPM)
  TrqCmd/1 -> Motor Torque Mapping and MCU Limiter/1(TrqCmd)
  Motor Torque Mapping and MCU Limiter/2(Torque) -> Power and Efficiency Estimator/1(Torque), Torque/1  "Motor_Torque(Nm)"
  Voltage/1 -> Power and Efficiency Estimator/2(Voltage)
  Power and Efficiency Estimator/1(Efficiency) -> Terminator/1  "Motor_Efficiency(%)"
  Power and Efficiency Estimator/2(PowerOutput) -> Terminator1/1  "Motor_P_output(kW)"
  Power and Efficiency Estimator/3(PowerConsume) -> Terminator2/1  "System_P_consume(kW)"
  Motor Torque Mapping and MCU Limiter/1(TrqLimit) -> TrqLimit/1
  Power and Efficiency Estimator/4(CurrentConsume) -> Current/1

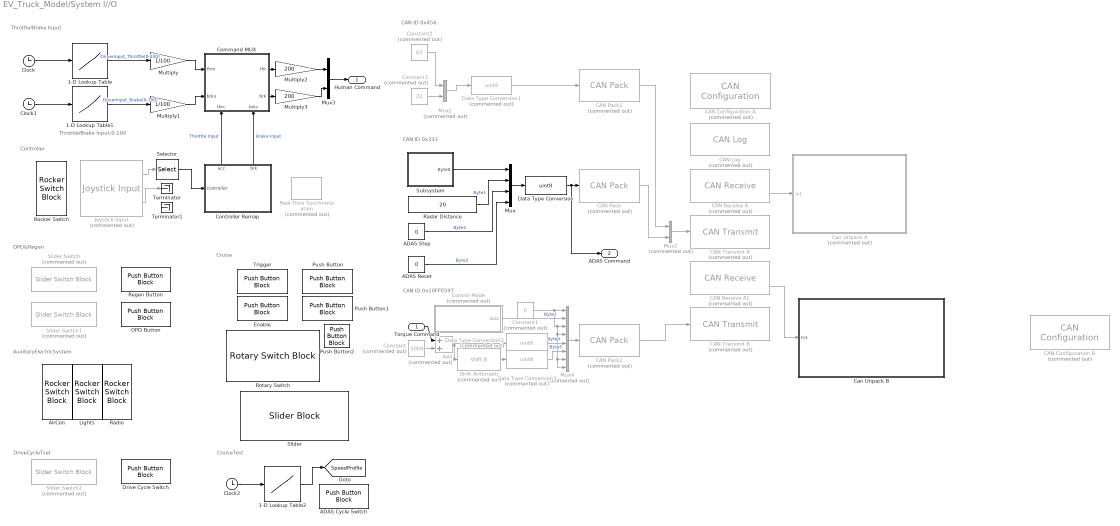
== system EV_Truck_Model/System I//O ==
  note: CruiseTest
  note: CAN ID 0x10FFE597
  note: AuxiliaryElectricSystem
  note: DriveCycleTset
  note: Cruise
  note: OPD&Regen
  note: Throttle/Brake Input:0-100
  note: Controller
  note: Throttle/Brake Input
  note: CAN ID 0x456
  note: CAN ID 0x333
  Torque Command : Inport
  1-D Lookup Table : Lookup_n-D  NumberOfTableDimensions=1  BreakpointsForDimension1=[0;10;24;25;35]  Table=[100;100;100;0;0]  InternalRulePriority=Speed  RndMeth=Simplest
  1-D Lookup Table1 : Lookup_n-D  NumberOfTableDimensions=1  BreakpointsForDimension1=[0 1 2 3 4 5 6 7 8 9 25 26 35]  Table=[0 0 0 0 0 0 0 0 0 0 0 100 100]  InternalRulePriority=Speed  RndMeth=Simplest
  1-D Lookup Table2 : Lookup_n-D  NumberOfTableDimensions=1  BreakpointsForDimension1=[0;20;21;30]  Table=[80;80;60;60]  InternalRulePriority=Speed  RndMeth=Simplest
  ADAS Cycle Switch : PushButtonBlock  ButtonText=ADASCycle  ButtonType=Latch  Icon=AdaptiveCruiseControl  IconAlignment=Center  IconColor=On  OffValue=0.000000
  ADAS Reset : Constant  Value=0  SampleTime=Sim_step
  ADAS Step : Constant  Value=0  SampleTime=Sim_step
  Add : Sum  Commented=on
  AirCon : RockerSwitchBlock
      settings: Values={{'Off', 'On'}, [0 2500]}
  CAN Configuration A : canlib/CAN Configuration  Commented=on  BlockHandle=1631.0001  Device=MathWorks Virtual 1 (Channel 1)  DeviceMenu=MathWorks Virtual 1 (Channel 1)  ObjConstructor=canChannel('MathWorks', 'Virtual 1', 1)  BusSpeed=500000  EnableBitParameters=off  AckMode=Normal
  CAN Configuration B : canlib/CAN Configuration  Commented=on  BlockHandle=1632.0001  Device=MathWorks Virtual 1 (Channel 2)  DeviceMenu=MathWorks Virtual 1 (Channel 2)  ObjConstructor=canChannel('MathWorks', 'Virtual 1', 2)  BusSpeed=250000  EnableBitParameters=off  AckMode=Normal
  CAN Log : canlib/CAN Log  Commented=on  BlockHandle=1633.0001  FullPathFileName=new.mat  FileName=new.mat  VariableName=ans  MaxNumMessages=10000  LogFrom=CAN Bus  DeviceMenu=MathWorks Virtual 1 (Channel 1)  Device=MathWorks Virtual 1 (Channel 1)  ObjConstructor=canChannel('MathWorks', 'Virtual 1', 1)  SampleTime=0.01
  CAN Pack : canmsglib/CAN Pack  Commented=on  MsgList=(none)  MsgName=CAN Msg  MsgIDType=Standard (11-bit identifier)  MsgIdentifier=0x333  MsgLength=8  Remote=off  ApplyMinMax=off  BusOutput=off  SignalInfo={}
      settings: LibrarySourceBlock=embeddedtargetslib/Host Communication/CAN Pack  DataFormat=raw data
  CAN Pack1 : canmsglib/CAN Pack  Commented=on  MsgList=(none)  MsgName=CAN Msg  MsgIDType=Standard (11-bit identifier)  MsgIdentifier=0x111  MsgLength=8  Remote=off  ApplyMinMax=off  BusOutput=off  SignalInfo={}
      settings: LibrarySourceBlock=embeddedtargetslib/Host Communication/CAN Pack  DataFormat=raw data
  CAN Pack2 : canmsglib/CAN Pack  Commented=on  MsgList=(none)  MsgName=CAN Msg  MsgIDType=Extended (29-bit identifier)  MsgIdentifier=0x10FFE597  MsgLength=8  Remote=off  ApplyMinMax=off  BusOutput=off  SignalInfo={}
      settings: LibrarySourceBlock=embeddedtargetslib/Host Communication/CAN Pack  DataFormat=raw data
  CAN Receive A : canlib/CAN Receive  Commented=on  BlockHandle=1643.0001  Device=MathWorks Virtual 1 (Channel 1)  DeviceMenu=MathWorks Virtual 1 (Channel 1)  ObjConstructor=canChannel('MathWorks', 'Virtual 1', 1)  EnableStandardIDsFilter=off  StdIDsCombo=Allow all  StandardIDs=0  EnableExtendedIDsFilter=off  ExtIDsCombo=Allow all  ExtendedIDs=0  SampleTime=0.01  MsgsPerTimestep=all  InternalFilterUpdateStatus=on  BusOutput=off
  CAN Receive A1 : canlib/CAN Receive  Commented=on  BlockHandle=1646.0001  Device=MathWorks Virtual 1 (Channel 2)  DeviceMenu=MathWorks Virtual 1 (Channel 2)  ObjConstructor=canChannel('MathWorks', 'Virtual 1', 2)  EnableStandardIDsFilter=off  StdIDsCombo=Allow all  StandardIDs=0  EnableExtendedIDsFilter=off  ExtIDsCombo=Allow all  ExtendedIDs=0  SampleTime=0.01  MsgsPerTimestep=all  InternalFilterUpdateStatus=on  BusOutput=off
  CAN Transmit A : canlib/CAN Transmit  Commented=on  BlockHandle=1649.0001  Device=MathWorks Virtual 1 (Channel 1)  DeviceMenu=MathWorks Virtual 1 (Channel 1)  ObjConstructor=canChannel('MathWorks', 'Virtual 1', 1)  EnableEventTransmit=off  EnablePeriodicTransmit=off  MessagePeriod=1.000
  CAN Transmit B : canlib/CAN Transmit  Commented=on  BlockHandle=1651.0001  Device=MathWorks Virtual 1 (Channel 2)  DeviceMenu=MathWorks Virtual 1 (Channel 2)  ObjConstructor=canChannel('MathWorks', 'Virtual 1', 2)  EnableEventTransmit=off  EnablePeriodicTransmit=off  MessagePeriod=1.000
  Can Unpack A : Subsystem  Commented=on
  "Can Unpack B " : Subsystem
  Clock : Clock
  Clock1 : Clock
  Clock2 : Clock
  Command MUX : Subsystem
      settings: PortSchema="{\"entries\":[{\"content\":{\"sides\":[{\"content\":{\"connectorIds\":[\"In1\",\"In2\"]},\"type\":\"ConnectorPlacement.EquallySpacedRectSide\",\"uuid\":\"b1935c73-897c-4bbd-a9a3-ce6c63cb0d14\"},{\"content\":{\"connectorIds\":[\"Out1\",\"Out2\"],\"side\":\"RIGHT\"},\"type\":\"ConnectorPlacement.EquallySpacedRectSide\",\"uuid\":\"1e8615e5-cfab-4f0e-9b90-e085b666e97c\"},{\"content\":{\"connectorIds\":[],\"side\":\"TOP\"},\"type\":\"ConnectorPlacement.EquallySpacedRectSide\",\"uuid\":\"bac445ec-0cf4-4989-9a3a-e58a2fcb7005\"},{\"content\":{\"connectorIds\":[\"In3\",\"In4\"],\"side\":\"BOTTOM\"},\"type\":\"ConnectorPlacement.EquallySpacedRectSide\",\"uuid\":\"4a63a39e-2584-4fad-a938-0a1bb95e689f\"}]},\"type\":\"ConnectorPlacement.EquallySpacedConnector\",\"uuid\":\"feb35536-eeb4-4e9a-8d0c-29f744dc8c34\"}],\"packageUris\":[\"http://schema.mathworks.com/mf0/Connector/R2020b\"],\"version\":\"1.0\"}"
  Constant : Constant  Commented=on  Value=5000
  Constant1 : Constant  Commented=on  Value=0
  Constant2 : Constant  Commented=on  Value=87
  Constant3 : Constant  Commented=on  Value=22
  Control Mode : Subsystem  Commented=on
  Controller Remap : Subsystem
      settings: PortSchema="{\"entries\":[{\"content\":{\"sides\":[{\"content\":{\"connectorIds\":[\"In1\"]},\"type\":\"ConnectorPlacement.EquallySpacedRectSide\",\"uuid\":\"1468438d-156c-432e-8c7c-7491ada65de9\"},{\"content\":{\"connectorIds\":[],\"side\":\"RIGHT\"},\"type\":\"ConnectorPlacement.EquallySpacedRectSide\",\"uuid\":\"87dc2bed-4c9f-4378-8a6c-52b79bf917c5\"},{\"content\":{\"connectorIds\":[\"Out1\",\"Out2\"],\"side\":\"TOP\"},\"type\":\"ConnectorPlacement.EquallySpacedRectSide\",\"uuid\":\"8fff4b6f-5f43-4315-8d94-3b434e664610\"}]},\"type\":\"ConnectorPlacement.EquallySpacedConnector\",\"uuid\":\"f17328f5-6980-4927-872b-ac8e2f5da073\"}],\"packageUris\":[\"http://schema.mathworks.com/mf0/Connector/R2020b\"],\"version\":\"1.0\"}"
  Data Type Conversion : DataTypeConversion  OutDataTypeStr=uint8  SaturateOnIntegerOverflow=off  RndMeth=Floor
  Data Type Conversion1 : DataTypeConversion  Commented=on  OutDataTypeStr=uint8  SaturateOnIntegerOverflow=off  RndMeth=Floor
  Data Type Conversion2 : DataTypeConversion  Commented=on  OutDataTypeStr=uint8  SaturateOnIntegerOverflow=off  RndMeth=Floor
  Data Type Conversion3 : DataTypeConversion  Commented=on  OutDataTypeStr=uint8  SaturateOnIntegerOverflow=off  RndMeth=Floor
  Drive Cycle Switch : PushButtonBlock  ButtonText=DriveCycle  ButtonType=Latch  Icon=AdaptiveCruiseControl  IconAlignment=Center  IconColor=On  OffValue=0.000000
  Enable : PushButtonBlock  ButtonText=Enable  ButtonType=Latch  Icon=CruiseControl  IconColor=On  OffValue=0.000000
  Joystick Input : vrlib/Joystick Input  Commented=on  joyid=1  adjustports=on  forcefeed=off
  Lights : RockerSwitchBlock
      settings: Values={{'Off', 'On'}, [0 250]}
  Multiply : Gain  Gain=1/100
  Multiply1 : Gain  Gain=1/100
  Multiply2 : Gain  Gain=200
  Multiply3 : Gain  Gain=200
  Mux : Mux
  Mux1 : Mux  Commented=on  Inputs=2
  Mux2 : Mux  Commented=on  Inputs=2
  Mux3 : Mux  Inputs=2
  Mux4 : Mux  Commented=on  Inputs=8
  OPD Button : PushButtonBlock  ButtonText=OPD  ButtonType=Latch  Icon=Engine  IconAlignment=Center  IconColor=On  OffValue=0.000000
  Push Button : PushButtonBlock  ButtonText=ADD  IconAlignment=Center  OffValue=0.000000
  Push Button1 : PushButtonBlock  ButtonText=MIN  OffValue=0.000000
  Push Button2 : PushButtonBlock  ButtonText=RESET  OffValue=0.000000
  Radar Distance : Constant  Value=20  SampleTime=Sim_step
  Radio : RockerSwitchBlock
      settings: Values={{'Off', 'On'}, [0 200]}
  Real-Time Synchronization : sldrtlib/Real-Time Synchronization  Commented=on  SampleTime=0.1  MaxMissedTicks=1000  ShowMissedTicks=off  YieldWhenWaiting=on
  Regen Button : PushButtonBlock  ButtonText=RGN  ButtonType=Latch  Icon=EcoMode  IconAlignment=Center  IconColor=On  OffValue=0.000000
  Rocker Switch : RockerSwitchBlock  LabelPosition=Hide
      settings: Values={{'Default', 'Controller'}, [0 1]}
  Rotary Switch : RotarySwitchBlock
      settings: Values={{'1 (Closest)', '2', '3', '4', '5 (Farthest)', 'Cruise Only'}, [1 2 3 4 5 0]}
  Selector : Selector  InputPortWidth=5  IndexOptions=Index vector (dialog)  Indices=3  OutputSizes=1
  Shift Arithmetic : ArithShift  Commented=on  BitShiftNumber=8
  Slider : SliderBlock  ScaleMax=20
  Slider Switch : SliderSwitchBlock  Commented=on
      settings: Values={{'Off', 'RGN On'}, [0 1]}
  Slider Switch1 : SliderSwitchBlock  Commented=on
      settings: Values={{'Off', 'OPD On'}, [0 1]}
  Slider Switch2 : SliderSwitchBlock  Commented=on
      settings: Values={{'Off', 'DriveCycle On'}, [0 1]}
  Subsystem : Subsystem
  Terminator : Terminator
  Terminator1 : Terminator
  Trigger : PushButtonBlock  ButtonText=On/Off  ButtonType=Latch  Icon=CruiseControl  IconColor=On  OffValue=0.000000
  Human Command : Outport
  ADAS Command : Outport  Port=2
  tag scope: SpeedProfile=global
  wires:
  Radar Distance/1 -> Mux/2  "Byte1"
  Mux2/1 -> CAN Transmit A/1
  Mux1/1 -> Data Type Conversion1/1
  CAN Pack/1 -> Mux2/2
  Constant3/1 -> Mux1/2
  CAN Pack1/1 -> Mux2/1
  Data Type Conversion1/1 -> CAN Pack1/1
  Mux/1 -> Data Type Conversion/1
  Constant2/1 -> Mux1/1
  Data Type Conversion/1 -> ADAS Command/1, CAN Pack/1
  1-D Lookup Table/1 -> Multiply/1  "DriverInput_Throttle(0-100)"
  1-D Lookup Table1/1 -> Multiply1/1  "DriverInput_Brake(0-100)"
  Clock/1 -> 1-D Lookup Table/1
  Clock1/1 -> 1-D Lookup Table1/1
  Multiply2/1 -> Mux3/1
  Mux3/1 -> Human Command/1
  Multiply3/1 -> Mux3/2
  ADAS Step/1 -> Mux/3  "Byte2"
  Joystick Input/1 -> Selector/1
  Joystick Input/2 -> Terminator/1
  ? -> Terminator1/1
  Selector/1 -> Controller Remap/1(controller)
  Controller Remap/1(acc) -> Command MUX/3(thrc)  "Throttle Input"
  Controller Remap/2(brk) -> Command MUX/4(brkc)  "Brake Input"
  Command MUX/1(thr) -> Multiply2/1
  Command MUX/2(brk) -> Multiply3/1
  CAN Receive A/2 -> Can Unpack A/1(In1)
  Subsystem/1(Byte0) -> Mux/1
  ADAS Reset/1 -> Mux/4  "Byte2"
  CAN Pack2/1 -> CAN Transmit B/1
  Torque Command/1 -> Add/1
  Constant/1 -> Add/2
  Add/1 -> Shift Arithmetic/1, Data Type Conversion2/1
  Shift Arithmetic/1 -> Data Type Conversion3/1
  Data Type Conversion2/1 -> Mux4/5  "Byte4"
  Data Type Conversion3/1 -> Mux4/6  "Byte5"
  Mux4/1 -> CAN Pack2/1
  CAN Receive A1/2 -> "Can Unpack B "/1(In1)
  Constant1/1 -> Mux4/8, Mux4/7, Mux4/4, Mux4/3, Mux4/1
  Control Mode/1(data) -> Mux4/2  "Byte1"
  Clock2/1 -> 1-D Lookup Table2/1
  1-D Lookup Table2/1 -> [SpeedProfile]
  Multiply/1 -> Command MUX/1(thro)
  Multiply1/1 -> Command MUX/2(brko)

== system EV_Truck_Model/VCU ==
  ADAS : Inport
  Speed : Inport  Port=2
  Human Command : Inport  Port=3
  Motor_RPM : Inport  Port=4
  SOC : Inport  Port=5
  TrqLimit : Inport  Port=6
  DriveCycle : Inport  Port=7
  Can Decode : Subsystem
  Demux : Demux  Outputs=2
  Demux1 : Demux  Outputs=3
  Remap Subsystem : Subsystem
      settings: PortSchema="{\"entries\":[{\"content\":{\"sides\":[{\"content\":{\"connectorIds\":[\"In1\",\"In2\",\"In3\",\"In4\",\"In5\",\"In6\",\"In7\",\"In8\",\"In9\",\"In10\",\"In11\",\"In12\",\"In13\"]},\"type\":\"ConnectorPlacement.EquallySpacedRectSide\",\"uuid\":\"be107167-99e2-43ad-9a51-0f5f1262385e\"},{\"content\":{\"connectorIds\":[\"Out1\",\"Out2\"],\"side\":\"RIGHT\"},\"type\":\"ConnectorPlacement.EquallySpacedRectSide\",\"uuid\":\"fdfeb49f-5ea0-44d9-8b7e-b7d2271ccf77\"},{\"content\":{\"connectorIds\":[\"In14\",\"In15\",\"In16\"],\"side\":\"TOP\"},\"type\":\"ConnectorPlacement.EquallySpacedRectSide\",\"uuid\":\"2920973c-97bd-4268-8e35-9bd469f1f48d\"}]},\"type\":\"ConnectorPlacement.EquallySpacedConnector\",\"uuid\":\"0f4b4950-7cc2-4123-a3fa-3acfc9cba22d\"}],\"packageUris\":[\"http://schema.mathworks.com/mf0/Connector/R2020b\"],\"version\":\"1.0\"}"
  TrqCmd : Outport
  BrakeCmd : Outport  Port=2
  wires:
  Demux/2 -> Remap Subsystem/10(Brake)
  TrqLimit/1 -> Remap Subsystem/13(TrqLimit)
  Motor_RPM/1 -> Remap Subsystem/11(Motor_RPM)
  SOC/1 -> Remap Subsystem/12(SOC)
  Remap Subsystem/1(TrqCmd) -> TrqCmd/1
  Human Command/1 -> Demux/1
  Demux/1 -> Remap Subsystem/9(Throttle)
  Remap Subsystem/2(BrakeCmd) -> BrakeCmd/1
  Speed/1 -> Remap Subsystem/8(Speed)
  ADAS/1 -> Can Decode/1(In1)
  Can Decode/1(ADAS on) -> Remap Subsystem/1(ADAS on)
  Can Decode/2(ADAS enable) -> Remap Subsystem/2(ADAS enable)
  Can Decode/3(ADAS add) -> Remap Subsystem/3(ADAS add)
  Can Decode/4(ADAS min) -> Remap Subsystem/4(ADAS min)
  Can Decode/5(Byte2) -> Remap Subsystem/5(ADAS mode)
  Demux1/2 -> Remap Subsystem/15(AccelCmd)
  Demux1/3 -> Remap Subsystem/16(DecelCmd)
  DriveCycle/1 -> Demux1/1
  Demux1/1 -> Remap Subsystem/14(DriveCycleEnable)
  Can Decode/6(ADAS_Distance) -> Remap Subsystem/6(ADAS_Distance)
  Can Decode/7(ADAS_Reset) -> Remap Subsystem/7(ADAS_Reset)

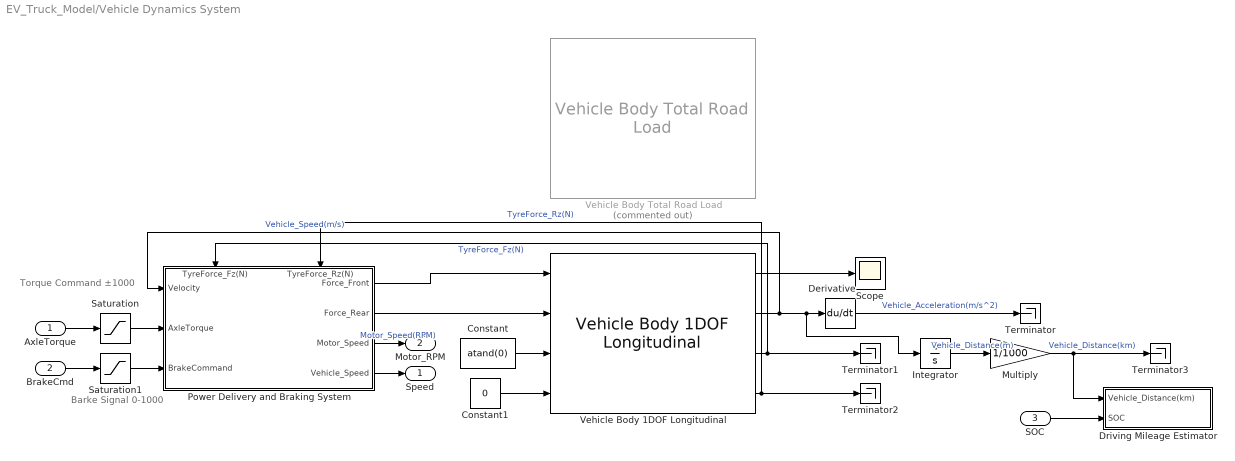
== system EV_Truck_Model/Vehicle Dynamics System ==
  note: Torque Command ±1000
  note: Barke Signal 0-1000
  AxleTorque : Inport
  BrakeCmd : Inport  Port=2
  SOC : Inport  Port=3
  Constant : Constant  Value=atand(0)
  Constant1 : Constant  Value=0
  Derivative : Derivative
  Driving Mileage Estimator : Subsystem
  Integrator : Integrator
  Multiply : Gain  Gain=1/1000
  Power Delivery and Braking System : Subsystem
      settings: PortSchema="{\"entries\":[{\"content\":{\"sides\":[{\"content\":{\"connectorIds\":[\"In1\",\"In2\",\"In3\"]},\"type\":\"ConnectorPlacement.EquallySpacedRectSide\",\"uuid\":\"3f1c80af-5c94-48ad-9185-0e33c89f3511\"},{\"content\":{\"connectorIds\":[\"Out1\",\"Out2\",\"Out3\",\"Out4\"],\"side\":\"RIGHT\"},\"type\":\"ConnectorPlacement.EquallySpacedRectSide\",\"uuid\":\"379fcf37-89af-420f-a2d0-f2806e8dc62c\"},{\"content\":{\"connectorIds\":[\"In4\",\"In5\"],\"side\":\"TOP\"},\"type\":\"ConnectorPlacement.EquallySpacedRectSide\",\"uuid\":\"c70b13aa-d05c-4901-b4cd-0d65f3ba777b\"}]},\"type\":\"ConnectorPlacement.EquallySpacedConnector\",\"uuid\":\"6166d447-7c37-43a4-a9e1-6b850883d776\"}],\"packageUris\":[\"http://schema.mathworks.com/mf0/Connector/R2020b\"],\"version\":\"1.0\"}"
  Saturation : Saturate  UpperLimit=1500  LowerLimit=-1500
  Saturation1 : Saturate  UpperLimit=1000  LowerLimit=0
  Scope : Scope
  Terminator{,1..3} (4 alike) : Terminator
  Vehicle Body 1DOF Longitudinal : autolibshared/Vehicle Body 1DOF Longitudinal  VariantControl=SL  extFMode=off  extMMode=off  extTamb=off  wind3D=off  aMode=2  NF=2  NR=4  m=Veh_mass  a=Veh_cog_fx  b=Veh_cog_rx  h=Veh_cog_h  Cd=.5  Cl=0  Cpm=0  Af=5.5  x_o=0  xdot_o=0  Pabs=101325  T=300  g=9.81
      settings: LibrarySourceBlock=vehdynlibeom/Vehicle Body 1DOF Longitudinal
  Vehicle Body Total Road Load : autolibshared/Vehicle Body Total Road Load  Commented=on  VariantControl=SL1dof  input_type=Force  aMode=2  m=1200  a=196  b=2.232  c=0.389  g=9.81  x_o=0  xdot_o=0
      settings: LibrarySourceBlock=vehdynlibeom/Vehicle Body Total Road Load
  Speed : Outport
  Motor_RPM : Outport  Port=2
  wires:
  AxleTorque/1 -> Saturation/1
  Power Delivery and Braking System/1(Force_Front) -> Vehicle Body 1DOF Longitudinal/1
  Power Delivery and Braking System/2(Force_Rear) -> Vehicle Body 1DOF Longitudinal/2
  Vehicle Body 1DOF Longitudinal/2 -> Power Delivery and Braking System/1(Velocity), Integrator/1, Derivative/1  "Vehicle_Speed(m/s)"
  Power Delivery and Braking System/3(Motor_Speed) -> Motor_RPM/1  "Motor_Speed(RPM)"
  Vehicle Body 1DOF Longitudinal/1 -> Scope/1
  Power Delivery and Braking System/4(Vehicle_Speed) -> Speed/1
  Constant/1 -> Vehicle Body 1DOF Longitudinal/3
  BrakeCmd/1 -> Saturation1/1
  Derivative/1 -> Terminator/1  "Vehicle_Acceleration(m/s^2)"
  Saturation/1 -> Power Delivery and Braking System/2(AxleTorque)
  Saturation1/1 -> Power Delivery and Braking System/3(BrakeCommand)
  Vehicle Body 1DOF Longitudinal/3 -> Terminator1/1, Power Delivery and Braking System/4(TyreForce_Fz(N))  "TyreForce_Fz(N)"
  Vehicle Body 1DOF Longitudinal/4 -> Terminator2/1, Power Delivery and Braking System/5(TyreForce_Rz(N))  "TyreForce_Rz(N)"
  Integrator/1 -> Multiply/1  "Vehicle_Distance(m)"
  Multiply/1 -> Driving Mileage Estimator/1(Vehicle_Distance(km)), Terminator3/1  "Vehicle_Distance(km)"
  SOC/1 -> Driving Mileage Estimator/2(SOC)
  Constant1/1 -> Vehicle Body 1DOF Longitudinal/4
